simulink model "grid_afe_n"  (R2026a)
settings: Solver=ode23tb  StopTime=simlength  FixedStep=tc  MaxStep=glb_time.tc
values from neighbouring files (symbols this model uses):
  afe_ctrl = ctrl_afe_setup(glb_time.ts_afe, grid_emu.omega_grid_nom)    [init_model.m]
  afe_pwm_phase_shift_mod1 = 0    [init_model.m]
  afe_pwm_phase_shift_mod2 = 0    [init_model.m]
  afe_pwm_phase_shift_mod3 = 0    [init_model.m]
  afe_pwm_phase_shift_mod4 = 0    [init_model.m]
  filters = setup_global_filters(glb_time.ts_afe, glb_time.ts_inv, glb_time.ts_dab, glb_time.tc)    [init_model.m]
  frt_data = frt_settings(test_index, test_subindex, asymmetric_error_type,      enable_frt_1, enable_frt_2, start_time_LVRT, deepPOSxi, deepPOSeta, deepNEGxi, deepNEGeta)    [init_model.m]
  glb_time = timing_setup(fpwm_afe, trgo_afe, fpwm_inv, trgo_inv, fpwm_single_phase_inv, trgo_single_phase_inv, fpwm_dab, trgo_dab,      fpwm_psfbc, trgo_psfbc, fpwm_isop_rail, trgo_isop_rail, fpwm_cllc, trgo_cllc, t_measure, tc_factor, tc_decimation, delay_pwm, dead_time_afe,      dead_time_inv, dead_time_single_phase_inv, dead_time_dab, dead_time_psfbc, dead_time_isop_rail, dead_time_cllc)    [init_model.m]
  grid_emu = grid_three_phase_emulator('Dyn11', delta_star, grid_nominal_power, application_voltage, us1, us2, fgrid,                  eq_grid_inductance, eq_grid_resistance, eta, ucc, i1m, p_iron, n1, n2, core_area, core_length, mur,                  up_xi_pu_ref, up_eta_pu_ref, un_xi_pu_ref, un_eta_pu_ref)    [init_model.m]
  i_react_pos_ref_2 = -ixi_ref_mod1*tan(acos(0.95))    [init_model.m]
  i_react_pos_ref_3 = ixi_ref_mod1*tan(acos(0.95))    [init_model.m]
  ixi_ref_mod1 = -0.85    [init_model.m]
  ixi_ref_mod2 = -0.85    [init_model.m]
  ixi_ref_mod3 = -0.85    [init_model.m]
  ixi_ref_mod4 = -0.85    [init_model.m]
  ki_align = 18    [init_model.m]
  kp_align = 0.25    [init_model.m]
  lim_down_align = -0.05    [init_model.m]
  lim_up_align = 0.05    [init_model.m]
  mavarage_filter_frequency_base_order = 2    [init_model.m]
  time_gain_afe_module_1 = 1.0002    [init_model.m]
  time_gain_afe_module_2 = 1.0015    [init_model.m]
  time_gain_afe_module_3 = 0.9988    [init_model.m]
  time_gain_afe_module_4 = 1.0020    (= 1.002)    [init_model.m]
  time_i_react_pos_ref_1 = start_time_LVRT + error_length + 0.335    [init_model.m]
  time_i_react_pos_ref_2 = time_i_react_pos_ref_1 + 0.5    (= 0.5)    [init_model.m]
  u_cm_comp_mod1 = 0    [init_model.m]
  u_cm_comp_mod2 = -1    [init_model.m]
  u_cm_comp_mod3 = -1    [init_model.m]
  u_cm_comp_mod4 = -1    [init_model.m]
undefined symbols (not defined in the file or in its folder): hwdata, magnitude
libraries: fl_lib x113, nesl_utility x75, moving_average_filter x40, moving_average_filter_cc x32, sl_discontinuities x12, linear_double_integrator_observer_ccaller x8, discrete_time_low_pass_filter x4, threephase_inductor_lib x4, dclink_for_two_levels x4, three_phase_pwm_modulator x4, three_phase_inverter_ideal_switch_based_model x4, three_phase_inverter_igbt_advanced_thermal_model x4
(part 15 of 19)

== system grid_afe_n/afe_abc_mod1/AFE_control/afe_control/current_ctrl/inner_current_ctrl/zero_current_ctrl/zero_sequence_current_ctrl ==
  iz : Inport
  1/Ti : Gain  Gain=afe_ctrl.kp_is_z  SaturateOnIntegerOverflow=on  OutDataTypeStr=Inherit: Same as input  ParamDataTypeStr=Inherit: Same as input
  Constant1 : Constant  Value=0
  Gain : Gain
  Saturation : Saturate  UpperLimit=1  LowerLimit=-1
  Sum1 : Sum  Inputs=+++  SaturateOnIntegerOverflow=on
  Sum2 : Sum  Inputs=-+  SaturateOnIntegerOverflow=on
  Sum3 : Sum  Inputs=-+  SaturateOnIntegerOverflow=on
  Unit Delay4 : UnitDelay  SampleTime=-1
  iz_tracking : Scope  NumInputPorts=3
      settings: ActiveDisplayYMinimum=-1  ActiveDisplayYMaximum=1  DataLoggingVariableName=ScopeData8
  kp : Gain  Gain=afe_ctrl.ki_is_z*glb_time.ts_afe  SaturateOnIntegerOverflow=on  OutDataTypeStr=Inherit: Same as input  ParamDataTypeStr=Inherit: Same as input
  ugamma_afe : Outport
  tag scope: iz_ctrl_out=scoped, iz_pu=scoped, iz_pu_ref=scoped
  wires:
  1/Ti/1 -> Sum1/1, Sum3/1
  kp/1 -> Sum1/2
  Sum3/1 -> Unit Delay4/1
  Unit Delay4/1 -> Sum1/3
  Constant1/1 -> [iz_pu_ref], iz_tracking/1, Sum2/2  "iz_pu_ref"
  iz/1 -> [iz_pu], iz_tracking/2, Sum2/1  "iz_pu"
  Sum2/1 -> kp/1, 1/Ti/1
  Sum1/1 -> Saturation/1
  Saturation/1 -> Gain/1, [iz_ctrl_out], iz_tracking/3, Sum3/2  "iz_ctrl_out"
  Gain/1 -> ugamma_afe/1

== system grid_afe_n/afe_abc_mod1/AFE_control/afe_control/grid_voltage_phase_lock_loops/FHT-PLL/pll_stageA/filter_and_transformation ==
  ug_a : Inport
  ug_b : Inport  Port=2
  ug_c : Inport  Port=3
  Bus Creator : BusCreator  Inputs=2
  Bus Creator1 : BusCreator  Inputs=3
  Bus Creator2 : BusCreator  Inputs=2
  Bus Creator3 : BusCreator  Inputs=3
  Bus Creator4 : BusCreator  Inputs=3
  FHTalpha : Subsystem
  FHTbeta : Subsystem
  FHTdqPLL : Scope  NumInputPorts=2
      settings: ActiveDisplayYMinimum=-1.5258214459194912  ActiveDisplayYMaximum=1.5258228058860459  DataLoggingVariableName=ScopeData12
  Gain : Gain  Gain=-1/2
  Gain1 : Gain  Gain=-1/2
  Sum : Sum  Inputs=|++
  Sum1 : Sum  Inputs=-+|
  To Workspace1 : ToWorkspace  VariableName=ugd_alpha_sim  SampleTime=-1
      settings: MaxDataPoints=glb_time.Ns_afe
  To Workspace2 : ToWorkspace  VariableName=ugd_beta_sim  SampleTime=-1
      settings: MaxDataPoints=glb_time.Ns_afe
  To Workspace3 : ToWorkspace  VariableName=u_fht_alpha_sim  SampleTime=-1
      settings: MaxDataPoints=glb_time.Ns_afe
  To Workspace4 : ToWorkspace  VariableName=v_fht_alpha_sim  SampleTime=-1
      settings: MaxDataPoints=glb_time.Ns_afe
  To Workspace5 : ToWorkspace  VariableName=u_fhtsr_alpha_sim  SampleTime=-1
      settings: MaxDataPoints=glb_time.Ns_afe
  To Workspace6 : ToWorkspace  VariableName=u_fhtsr_beta_sim  SampleTime=-1
      settings: MaxDataPoints=glb_time.Ns_afe
  To Workspace7 : ToWorkspace  VariableName=u_fht_beta_sim  SampleTime=-1
      settings: MaxDataPoints=glb_time.Ns_afe
  To Workspace8 : ToWorkspace  VariableName=v_fht_beta_sim  SampleTime=-1
      settings: MaxDataPoints=glb_time.Ns_afe
  To Workspace9 : ToWorkspace  VariableName=ugd_abc_grid_sim  SampleTime=-1
      settings: MaxDataPoints=glb_time.Ns_afe
  abc2alphabeta : MATLAB Function  TreatAsAtomicUnit=on
  grid_voltages : Scope  NumInputPorts=3
      settings: ActiveDisplayYMinimum=-1.3618303835391998  ActiveDisplayYMaximum=1.3331545889377594  DataLoggingVariableName=ScopeData13
  ug_alpha : Outport  VectorParamsAs1DForOutWhenUnconnected=off
  ug_beta : Outport  Port=2  VectorParamsAs1DForOutWhenUnconnected=off
  wires:
  ug_b/1 -> Bus Creator3/2, grid_voltages/2, abc2alphabeta/2(b)  "ugd_b"
  ug_c/1 -> Bus Creator3/3, grid_voltages/3, abc2alphabeta/3(c)  "ugd_c"
  ug_a/1 -> Bus Creator3/1, grid_voltages/1, abc2alphabeta/1(a)  "ugd_a"
  abc2alphabeta/1(alpha) -> To Workspace1/1, FHTalpha/1(u), Bus Creator4/1  "u_grid_alpha"
  abc2alphabeta/2(beta) -> FHTbeta/1(u), To Workspace2/1, Bus Creator1/1  "u_grid_beta"
  FHTalpha/1(ud_hat) -> To Workspace3/1, Bus Creator/1, Sum/1  "u_fht_alpha"
  Sum/1 -> Gain/1
  FHTbeta/1(ud_hat) -> Sum1/2, To Workspace7/1, Bus Creator2/1  "u_fht_beta"
  Sum1/1 -> Gain1/1
  Gain1/1 -> Bus Creator1/3, To Workspace6/1, ug_beta/1  "u_fhtsr_beta"
  Gain/1 -> Bus Creator4/3, To Workspace5/1, ug_alpha/1  "u_fhtsr_alpha"
  FHTbeta/2(uq_hat) -> Sum/2, To Workspace8/1, Bus Creator2/2  "v_fht_beta"
  FHTalpha/2(uq_hat) -> Sum1/1, To Workspace4/1, Bus Creator/2  "v_fht_alpha"
  Bus Creator1/1 -> FHTdqPLL/2
  Bus Creator4/1 -> FHTdqPLL/1
  Bus Creator/1 -> Bus Creator4/2  "FHTalpha"
  Bus Creator2/1 -> Bus Creator1/2  "FHTbeta"
  Bus Creator3/1 -> To Workspace9/1

== system grid_afe_n/afe_abc_mod1/AFE_control/afe_control/grid_voltage_phase_lock_loops/FHT-PLL/pll_stageA/sequences ==
  u_grid_alpha : Inport
  u_grid_beta : Inport  Port=2
  phase_angle : Inport  Port=3
  alphabeta2xieta : MATLAB Function  TreatAsAtomicUnit=on
  u_grid_xi : Outport
  u_grid_eta : Outport  Port=2
  wires:
  alphabeta2xieta/1(xi) -> u_grid_xi/1  "u_grid_xi"
  alphabeta2xieta/2(eta) -> u_grid_eta/1  "u_grid_eta"
  u_grid_alpha/1 -> alphabeta2xieta/1(alpha)  "u_grid_alpha"
  u_grid_beta/1 -> alphabeta2xieta/2(beta)  "u_grid_beta"
  phase_angle/1 -> alphabeta2xieta/3(gamma)  "phase_angle"

== system grid_afe_n/afe_abc_mod1/AFE_control/afe_control/grid_voltage_phase_lock_loops/FHT-PLL/pll_stageB/double_integrator_observer ==
  theta : Inport
  Gain : Gain  Gain=afe_ctrl.di_obs.Ldso  Multiplication=Matrix(K*u)
  Gain1 : Gain  Gain=afe_ctrl.di_obs.Adso  Multiplication=Matrix(K*u)
  Gain2 : Gain  Gain=afe_ctrl.di_obs.Cso  Multiplication=Matrix(K*u)
  Selector : Selector  InputPortWidth=2  IndexOptions=Index vector (dialog)  Indices=2  OutputSizes=1
  Sum : Sum  Inputs=-+|
  Sum1 : Sum  Inputs=|++
  Unit Delay : UnitDelay  SampleTime=-1
  bounder1 : MATLAB Function  TreatAsAtomicUnit=on
  bounder2 : MATLAB Function  TreatAsAtomicUnit=on
  omega_hat : Outport
  wires:
  Gain/1 -> Sum1/1
  Selector/1 -> omega_hat/1
  Gain2/1 -> bounder2/1(u)  "theta_hat"
  Gain1/1 -> Sum1/2
  Sum1/1 -> Unit Delay/1
  Sum/1 -> bounder1/1(u)  "e"
  Unit Delay/1 -> Gain1/1, Selector/1, Gain2/1
  theta/1 -> Sum/2  "theta"
  bounder1/1(y) -> Gain/1
  bounder2/1(y) -> Sum/1  "theta_hat_bounded"

== system grid_afe_n/afe_abc_mod1/AFE_control/afe_control/grid_voltage_phase_lock_loops/FHT-PLL_simulink/pll_stageA/filter_and_transformation ==
  ug_a : Inport
  ug_b : Inport  Port=2
  ug_c : Inport  Port=3
  Bus Creator : BusCreator  Inputs=2
  Bus Creator1 : BusCreator  Inputs=3
  Bus Creator2 : BusCreator  Inputs=2
  Bus Creator4 : BusCreator  Inputs=3
  FHTalpha : Subsystem
  FHTbeta : Subsystem
  FHTdqPLL : Scope  NumInputPorts=2
      settings: ActiveDisplayYMinimum=-1.5258214459194912  ActiveDisplayYMaximum=1.5258228058860459  DataLoggingVariableName=ScopeData12
  Gain : Gain  Gain=-1/2
  Gain1 : Gain  Gain=-1/2
  Sum : Sum  Inputs=|++
  Sum1 : Sum  Inputs=-+|
  abc2alphabeta : MATLAB Function  TreatAsAtomicUnit=on
  grid_voltages : Scope  NumInputPorts=3
      settings: ActiveDisplayYMinimum=-1.3618303835391998  ActiveDisplayYMaximum=1.3331545889377594  DataLoggingVariableName=ScopeData13
  ug_alpha : Outport  VectorParamsAs1DForOutWhenUnconnected=off
  ug_beta : Outport  Port=2  VectorParamsAs1DForOutWhenUnconnected=off
  wires:
  Bus Creator2/1 -> Bus Creator1/2  "FHTbeta"
  Bus Creator/1 -> Bus Creator4/2  "FHTalpha"
  Bus Creator4/1 -> FHTdqPLL/1
  Bus Creator1/1 -> FHTdqPLL/2
  FHTalpha/2(ubeta) -> Bus Creator/2, Sum1/1  "v_fht_alpha"
  FHTbeta/2(ubeta) -> Bus Creator2/2, Sum/2  "v_fht_beta"
  Gain/1 -> ug_alpha/1, Bus Creator4/3  "u_fhtsr_alpha"
  Gain1/1 -> ug_beta/1, Bus Creator1/3  "u_fhtsr_beta"
  Sum1/1 -> Gain1/1
  FHTbeta/1(ualpha) -> Bus Creator2/1, Sum1/2  "u_fht_beta"
  Sum/1 -> Gain/1
  FHTalpha/1(ualpha) -> Sum/1, Bus Creator/1  "u_fht_alpha"
  abc2alphabeta/2(beta) -> FHTbeta/1(u), Bus Creator1/1  "u_grid_beta"
  abc2alphabeta/1(alpha) -> FHTalpha/1(u), Bus Creator4/1  "u_grid_alpha"
  ug_a/1 -> abc2alphabeta/1(a), grid_voltages/1  "ugd_a"
  ug_c/1 -> abc2alphabeta/3(c), grid_voltages/3  "ugd_c"
  ug_b/1 -> abc2alphabeta/2(b), grid_voltages/2  "ugd_b"

== system grid_afe_n/afe_abc_mod1/AFE_control/afe_control/grid_voltage_phase_lock_loops/FHT-PLL_simulink/pll_stageA/sequences ==
  u_grid_alpha : Inport
  u_grid_beta : Inport  Port=2
  phase_angle : Inport  Port=3
  alphabeta2xieta : MATLAB Function  TreatAsAtomicUnit=on
  u_grid_xi : Outport
  u_grid_eta : Outport  Port=2
  wires:
  phase_angle/1 -> alphabeta2xieta/3(gamma)  "phase_angle"
  u_grid_beta/1 -> alphabeta2xieta/2(beta)  "u_grid_beta"
  u_grid_alpha/1 -> alphabeta2xieta/1(alpha)  "u_grid_alpha"
  alphabeta2xieta/2(eta) -> u_grid_eta/1  "u_grid_eta"
  alphabeta2xieta/1(xi) -> u_grid_xi/1  "u_grid_xi"

== system grid_afe_n/afe_abc_mod1/AFE_control/afe_control/grid_voltage_phase_lock_loops/FHT-PLL_simulink/pll_stageB/double_integrator_observer ==
  theta : Inport
  Gain : Gain  Gain=afe_ctrl.di_obs.Ldso  Multiplication=Matrix(K*u)
  Gain1 : Gain  Gain=afe_ctrl.di_obs.Adso  Multiplication=Matrix(K*u)
  Gain2 : Gain  Gain=afe_ctrl.di_obs.Cso  Multiplication=Matrix(K*u)
  Selector : Selector  InputPortWidth=2  IndexOptions=Index vector (dialog)  Indices=2  OutputSizes=1
  Sum : Sum  Inputs=-+|
  Sum1 : Sum  Inputs=|++
  Unit Delay : UnitDelay  SampleTime=-1
  bounder1 : MATLAB Function  TreatAsAtomicUnit=on
  bounder2 : MATLAB Function  TreatAsAtomicUnit=on
  omega_hat : Outport
  wires:
  bounder2/1(y) -> Sum/1  "theta_hat_bounded"
  bounder1/1(y) -> Gain/1
  theta/1 -> Sum/2  "theta"
  Unit Delay/1 -> Gain2/1, Selector/1, Gain1/1
  Sum/1 -> bounder1/1(u)  "e"
  Sum1/1 -> Unit Delay/1
  Gain1/1 -> Sum1/2
  Gain2/1 -> bounder2/1(u)  "theta_hat"
  Selector/1 -> omega_hat/1
  Gain/1 -> Sum1/1

== system grid_afe_n/afe_abc_mod1/AFE_control/afe_control/grid_voltage_phase_lock_loops/dq_pll/pll_stageA/mormalization_and_transformation ==
  ug_a : Inport
  ug_b : Inport  Port=2
  ug_c : Inport  Port=3
  abc2alphabeta : MATLAB Function  TreatAsAtomicUnit=on
  ug_alpha : Outport  VectorParamsAs1DForOutWhenUnconnected=off
  ug_beta : Outport  Port=2  VectorParamsAs1DForOutWhenUnconnected=off
  wires:
  abc2alphabeta/2(beta) -> ug_beta/1  "u_grid_beta"
  abc2alphabeta/1(alpha) -> ug_alpha/1  "u_grid_alpha"
  ug_a/1 -> abc2alphabeta/1(a)
  ug_b/1 -> abc2alphabeta/2(b)
  ug_c/1 -> abc2alphabeta/3(c)

== system grid_afe_n/afe_abc_mod1/AFE_control/afe_control/grid_voltage_phase_lock_loops/dq_pll/pll_stageA/sequences ==
  u_grid_alpha : Inport
  u_grid_beta : Inport  Port=2
  gamma_grid : Inport  Port=3
  Terminator : Terminator
  Terminator1 : Terminator
  alphabeta2xieta : Subsystem
  u_grid_pos_xi : Outport
  u_grid_pos_eta : Outport  Port=2
  wires:
  alphabeta2xieta/1(xi) -> u_grid_pos_xi/1  "u_grid_pos_xi"
  alphabeta2xieta/2(eta) -> u_grid_pos_eta/1  "u_grid_pos_eta"
  u_grid_alpha/1 -> alphabeta2xieta/1(alpha)  "u_grid_alpha"
  u_grid_beta/1 -> alphabeta2xieta/2(beta)  "u_grid_beta"
  gamma_grid/1 -> alphabeta2xieta/3(gamma)  "phase_grid"
  alphabeta2xieta/3(Out3) -> Terminator/1  "neg_xi"
  alphabeta2xieta/4(Out4) -> Terminator1/1  "neg_eta"

== system grid_afe_n/afe_abc_mod1/AFE_control/afe_control/grid_voltage_phase_lock_loops/dq_pll/pll_stageB/double_integrator_observer ==
  phase : Inport
  Gain : Gain  Gain=afe_ctrl.di_obs.Ldso  Multiplication=Matrix(K*u)
  Gain1 : Gain  Gain=afe_ctrl.di_obs.Adso  Multiplication=Matrix(K*u)
  Gain2 : Gain  Gain=afe_ctrl.di_obs.Cso  Multiplication=Matrix(K*u)
  Selector : Selector  InputPortWidth=2  IndexOptions=Index vector (dialog)  Indices=2  OutputSizes=1
  Sum : Sum  Inputs=-+|
  Sum1 : Sum  Inputs=|++
  Unit Delay : UnitDelay  SampleTime=-1
  bounder1 : MATLAB Function  TreatAsAtomicUnit=on
  bounder2 : MATLAB Function  TreatAsAtomicUnit=on
  omega_hat : Outport
  wires:
  Gain/1 -> Sum1/1
  Selector/1 -> omega_hat/1
  Gain2/1 -> bounder2/1(u)  "theta_hat"
  Gain1/1 -> Sum1/2
  Sum1/1 -> Unit Delay/1
  Sum/1 -> bounder1/1(u)  "e"
  Unit Delay/1 -> Gain1/1, Selector/1, Gain2/1
  phase/1 -> Sum/2  "phase"
  bounder1/1(y) -> Gain/1  "e_bounded"
  bounder2/1(y) -> Sum/1  "theta_hat_bounded"

== system grid_afe_n/afe_abc_mod1/AFE_control/afe_control/grid_voltage_phase_lock_loops/dq_pll/pll_stageB/scheduled-p-gain ==
  In1 : Inport
  Switch : Switch  Criteria=u2 > Threshold  Threshold=0.5  SaturateOnIntegerOverflow=off  InputSameDT=off
  kp1 : Gain  Gain=afe_ctrl.pll_p  SaturateOnIntegerOverflow=on  OutDataTypeStr=Inherit: Same as input  ParamDataTypeStr=Inherit: Same as input
  kp3 : Gain  Gain=afe_ctrl.pll_p_frt  SaturateOnIntegerOverflow=on  OutDataTypeStr=Inherit: Same as input  ParamDataTypeStr=Inherit: Same as input
  Out2 : Outport
  wires:
  kp3/1 -> Switch/1
  kp1/1 -> Switch/3
  [frt_active] -> Switch/2
  In1/1 -> kp1/1, kp3/1
  Switch/1 -> Out2/1

== system grid_afe_n/afe_abc_mod2/AFE_control/afe_control/current_ctrl/inner_current_ctrl/zero_current_ctrl/antiwind_up ==
  d_abc : Inport
  Add : Sum
  Bus Creator : BusCreator  Inputs=3
  Constant : Constant  Value=0
  Demux1 : Demux  Outputs=3
  MATLAB Function1 : MATLAB Function  TreatAsAtomicUnit=on
  MATLAB Function2 : MATLAB Function  TreatAsAtomicUnit=on
  Terminator : Terminator
  Unit Delay1 : UnitDelay  SampleTime=-1
  Unit Delay4 : UnitDelay  SampleTime=-1
  Unit Delay5 : UnitDelay  SampleTime=-1
  afe_ictrl_out/afe_ictrl_ff : Scope  NumInputPorts=3
      settings: ActiveDisplayYMinimum=-1.3378870671178225  ActiveDisplayYMaximum=1.3487234823223584  DataLoggingVariableName=ScopeData4
  anti_wind_up : Subsystem
  ualpha_afe : Outport
  ubeta_afe : Outport  Port=2
  wires:
  Constant/1 -> Add/2
  MATLAB Function2/3(gamma) -> Terminator/1  "u_gamma"
  Unit Delay5/1 -> ubeta_afe/1, anti_wind_up/2(beta)  "ubeta_afe"
  MATLAB Function2/2(beta) -> Unit Delay5/1  "u_beta"
  Unit Delay4/1 -> ualpha_afe/1, anti_wind_up/1(alpha)  "ualpha_afe"
  MATLAB Function2/1(alpha) -> Unit Delay4/1  "u_alpha"
  MATLAB Function1/2(dbs) -> Bus Creator/2, MATLAB Function2/2(b)  "dbs"
  Add/1 -> Demux1/1  "d_abc_sum"
  Demux1/1 -> MATLAB Function1/1(da)  "da"
  anti_wind_up/1(scaling) -> MATLAB Function1/4(scaling)
  Unit Delay1/1 -> afe_ictrl_out/afe_ictrl_ff/3  "u_grid_ff_abc_mod1"
  Bus Creator/1 -> afe_ictrl_out/afe_ictrl_ff/1  "ds_abc"
  Demux1/3 -> MATLAB Function1/3(dc)  "dc"
  Demux1/2 -> MATLAB Function1/2(db)  "db"
  [v_grid_ff_abc] -> Unit Delay1/1
  MATLAB Function1/3(dcs) -> Bus Creator/3, MATLAB Function2/3(c)  "dcs"
  d_abc/1 -> afe_ictrl_out/afe_ictrl_ff/2, Add/1
  MATLAB Function1/1(das) -> Bus Creator/1, MATLAB Function2/1(a)  "das"

== system grid_afe_n/afe_abc_mod2/AFE_control/afe_control/current_ctrl/inner_current_ctrl/zero_current_ctrl/iz ==
  Demux : Demux  Outputs=3
  Gain : Gain  Gain=1/3
  Sum : Sum  Inputs=+++
  iz : Outport
  wires:
  Gain/1 -> iz/1
  Demux/2 -> Sum/2  "is_b"
  Demux/3 -> Sum/3  "is_c"
  [isd_abc_pu] -> Demux/1
  Demux/1 -> Sum/1  "is_a"
  Sum/1 -> Gain/1

== system grid_afe_n/afe_abc_mod2/AFE_control/afe_control/current_ctrl/inner_current_ctrl/zero_current_ctrl/zero_sequence_current_ctrl ==
  iz : Inport
  1/Ti : Gain  Gain=afe_ctrl.kp_is_z  SaturateOnIntegerOverflow=on  OutDataTypeStr=Inherit: Same as input  ParamDataTypeStr=Inherit: Same as input
  Constant1 : Constant  Value=0
  Gain : Gain
  Saturation : Saturate  UpperLimit=1  LowerLimit=-1
  Sum1 : Sum  Inputs=+++  SaturateOnIntegerOverflow=on
  Sum2 : Sum  Inputs=-+  SaturateOnIntegerOverflow=on
  Sum3 : Sum  Inputs=-+  SaturateOnIntegerOverflow=on
  Unit Delay4 : UnitDelay  SampleTime=-1
  iz_tracking : Scope  NumInputPorts=3
      settings: ActiveDisplayYMinimum=-1  ActiveDisplayYMaximum=1  DataLoggingVariableName=ScopeData8
  kp : Gain  Gain=afe_ctrl.ki_is_z*glb_time.ts_afe  SaturateOnIntegerOverflow=on  OutDataTypeStr=Inherit: Same as input  ParamDataTypeStr=Inherit: Same as input
  ugamma_afe : Outport
  tag scope: iz_ctrl_out=scoped, iz_pu=scoped, iz_pu_ref=scoped
  wires:
  Gain/1 -> ugamma_afe/1
  Saturation/1 -> Sum3/2, iz_tracking/3, [iz_ctrl_out], Gain/1  "iz_ctrl_out"
  Sum1/1 -> Saturation/1
  Sum2/1 -> 1/Ti/1, kp/1
  iz/1 -> Sum2/1, iz_tracking/2, [iz_pu]  "iz_pu"
  Constant1/1 -> Sum2/2, iz_tracking/1, [iz_pu_ref]  "iz_pu_ref"
  Unit Delay4/1 -> Sum1/3
  Sum3/1 -> Unit Delay4/1
  kp/1 -> Sum1/2
  1/Ti/1 -> Sum3/1, Sum1/1

== system grid_afe_n/afe_abc_mod2/AFE_control/afe_control/grid_voltage_phase_lock_loops/FHT-PLL/pll_stageA/filter_and_transformation ==
  ug_a : Inport
  ug_b : Inport  Port=2
  ug_c : Inport  Port=3
  Bus Creator : BusCreator  Inputs=2
  Bus Creator1 : BusCreator  Inputs=3
  Bus Creator2 : BusCreator  Inputs=2
  Bus Creator3 : BusCreator  Inputs=3
  Bus Creator4 : BusCreator  Inputs=3
  FHTalpha : Subsystem
  FHTbeta : Subsystem
  FHTdqPLL : Scope  NumInputPorts=2
      settings: ActiveDisplayYMinimum=-1.5258214459194912  ActiveDisplayYMaximum=1.5258228058860459  DataLoggingVariableName=ScopeData12
  Gain : Gain  Gain=-1/2
  Gain1 : Gain  Gain=-1/2
  Sum : Sum  Inputs=|++
  Sum1 : Sum  Inputs=-+|
  To Workspace1 : ToWorkspace  VariableName=ugd_alpha_sim  SampleTime=-1
      settings: MaxDataPoints=glb_time.Ns_afe
  To Workspace2 : ToWorkspace  VariableName=ugd_beta_sim  SampleTime=-1
      settings: MaxDataPoints=glb_time.Ns_afe
  To Workspace3 : ToWorkspace  VariableName=u_fht_alpha_sim  SampleTime=-1
      settings: MaxDataPoints=glb_time.Ns_afe
  To Workspace4 : ToWorkspace  VariableName=v_fht_alpha_sim  SampleTime=-1
      settings: MaxDataPoints=glb_time.Ns_afe
  To Workspace5 : ToWorkspace  VariableName=u_fhtsr_alpha_sim  SampleTime=-1
      settings: MaxDataPoints=glb_time.Ns_afe
  To Workspace6 : ToWorkspace  VariableName=u_fhtsr_beta_sim  SampleTime=-1
      settings: MaxDataPoints=glb_time.Ns_afe
  To Workspace7 : ToWorkspace  VariableName=u_fht_beta_sim  SampleTime=-1
      settings: MaxDataPoints=glb_time.Ns_afe
  To Workspace8 : ToWorkspace  VariableName=v_fht_beta_sim  SampleTime=-1
      settings: MaxDataPoints=glb_time.Ns_afe
  To Workspace9 : ToWorkspace  VariableName=ugd_abc_grid_sim  SampleTime=-1
      settings: MaxDataPoints=glb_time.Ns_afe
  abc2alphabeta : MATLAB Function  TreatAsAtomicUnit=on
  grid_voltages : Scope  NumInputPorts=3
      settings: ActiveDisplayYMinimum=-1.3618303835391998  ActiveDisplayYMaximum=1.3331545889377594  DataLoggingVariableName=ScopeData13
  ug_alpha : Outport  VectorParamsAs1DForOutWhenUnconnected=off
  ug_beta : Outport  Port=2  VectorParamsAs1DForOutWhenUnconnected=off
  wires:
  Bus Creator3/1 -> To Workspace9/1
  Bus Creator2/1 -> Bus Creator1/2  "FHTbeta"
  Bus Creator/1 -> Bus Creator4/2  "FHTalpha"
  Bus Creator4/1 -> FHTdqPLL/1
  Bus Creator1/1 -> FHTdqPLL/2
  FHTalpha/2(uq_hat) -> Bus Creator/2, To Workspace4/1, Sum1/1  "v_fht_alpha"
  FHTbeta/2(uq_hat) -> Bus Creator2/2, To Workspace8/1, Sum/2  "v_fht_beta"
  Gain/1 -> ug_alpha/1, To Workspace5/1, Bus Creator4/3  "u_fhtsr_alpha"
  Gain1/1 -> ug_beta/1, To Workspace6/1, Bus Creator1/3  "u_fhtsr_beta"
  Sum1/1 -> Gain1/1
  FHTbeta/1(ud_hat) -> Bus Creator2/1, To Workspace7/1, Sum1/2  "u_fht_beta"
  Sum/1 -> Gain/1
  FHTalpha/1(ud_hat) -> Sum/1, Bus Creator/1, To Workspace3/1  "u_fht_alpha"
  abc2alphabeta/2(beta) -> Bus Creator1/1, To Workspace2/1, FHTbeta/1(u)  "u_grid_beta"
  abc2alphabeta/1(alpha) -> Bus Creator4/1, FHTalpha/1(u), To Workspace1/1  "u_grid_alpha"
  ug_a/1 -> abc2alphabeta/1(a), grid_voltages/1, Bus Creator3/1  "ugd_a"
  ug_c/1 -> abc2alphabeta/3(c), grid_voltages/3, Bus Creator3/3  "ugd_c"
  ug_b/1 -> abc2alphabeta/2(b), grid_voltages/2, Bus Creator3/2  "ugd_b"

== system grid_afe_n/afe_abc_mod2/AFE_control/afe_control/grid_voltage_phase_lock_loops/FHT-PLL/pll_stageA/sequences ==
  u_grid_alpha : Inport
  u_grid_beta : Inport  Port=2
  phase_angle : Inport  Port=3
  alphabeta2xieta : MATLAB Function  TreatAsAtomicUnit=on
  u_grid_xi : Outport
  u_grid_eta : Outport  Port=2
  wires:
  phase_angle/1 -> alphabeta2xieta/3(gamma)  "phase_angle"
  u_grid_beta/1 -> alphabeta2xieta/2(beta)  "u_grid_beta"
  u_grid_alpha/1 -> alphabeta2xieta/1(alpha)  "u_grid_alpha"
  alphabeta2xieta/2(eta) -> u_grid_eta/1  "u_grid_eta"
  alphabeta2xieta/1(xi) -> u_grid_xi/1  "u_grid_xi"

== system grid_afe_n/afe_abc_mod2/AFE_control/afe_control/grid_voltage_phase_lock_loops/FHT-PLL/pll_stageB/double_integrator_observer ==
  theta : Inport
  Gain : Gain  Gain=afe_ctrl.di_obs.Ldso  Multiplication=Matrix(K*u)
  Gain1 : Gain  Gain=afe_ctrl.di_obs.Adso  Multiplication=Matrix(K*u)
  Gain2 : Gain  Gain=afe_ctrl.di_obs.Cso  Multiplication=Matrix(K*u)
  Selector : Selector  InputPortWidth=2  IndexOptions=Index vector (dialog)  Indices=2  OutputSizes=1
  Sum : Sum  Inputs=-+|
  Sum1 : Sum  Inputs=|++
  Unit Delay : UnitDelay  SampleTime=-1
  bounder1 : MATLAB Function  TreatAsAtomicUnit=on
  bounder2 : MATLAB Function  TreatAsAtomicUnit=on
  omega_hat : Outport
  wires:
  bounder2/1(y) -> Sum/1  "theta_hat_bounded"
  bounder1/1(y) -> Gain/1
  theta/1 -> Sum/2  "theta"
  Unit Delay/1 -> Gain2/1, Selector/1, Gain1/1
  Sum/1 -> bounder1/1(u)  "e"
  Sum1/1 -> Unit Delay/1
  Gain1/1 -> Sum1/2
  Gain2/1 -> bounder2/1(u)  "theta_hat"
  Selector/1 -> omega_hat/1
  Gain/1 -> Sum1/1

== system grid_afe_n/afe_abc_mod2/AFE_control/afe_control/grid_voltage_phase_lock_loops/FHT-PLL_simulink/pll_stageA/filter_and_transformation ==
  ug_a : Inport
  ug_b : Inport  Port=2
  ug_c : Inport  Port=3
  Bus Creator : BusCreator  Inputs=2
  Bus Creator1 : BusCreator  Inputs=3
  Bus Creator2 : BusCreator  Inputs=2
  Bus Creator4 : BusCreator  Inputs=3
  FHTalpha : Subsystem
  FHTbeta : Subsystem
  FHTdqPLL : Scope  NumInputPorts=2
      settings: ActiveDisplayYMinimum=-1.4370650300424566  ActiveDisplayYMaximum=1.3792236516012133  DataLoggingVariableName=ScopeData12
  Gain : Gain  Gain=-1/2
  Gain1 : Gain  Gain=-1/2
  Sum : Sum  Inputs=|++
  Sum1 : Sum  Inputs=-+|
  abc2alphabeta : MATLAB Function  TreatAsAtomicUnit=on
  grid_voltages : Scope  NumInputPorts=3
      settings: ActiveDisplayYMinimum=-1.3620119839906693  ActiveDisplayYMaximum=1.3591613322496414  DataLoggingVariableName=ScopeData13
  ug_alpha : Outport  VectorParamsAs1DForOutWhenUnconnected=off
  ug_beta : Outport  Port=2  VectorParamsAs1DForOutWhenUnconnected=off
  wires:
  Bus Creator2/1 -> Bus Creator1/2  "FHTbeta"
  Bus Creator/1 -> Bus Creator4/2  "FHTalpha"
  Bus Creator4/1 -> FHTdqPLL/1
  Bus Creator1/1 -> FHTdqPLL/2
  FHTalpha/2(ubeta) -> Bus Creator/2, Sum1/1  "v_fht_alpha"
  FHTbeta/2(ubeta) -> Bus Creator2/2, Sum/2  "v_fht_beta"
  Gain/1 -> ug_alpha/1, Bus Creator4/3  "u_fhtsr_alpha"
  Gain1/1 -> ug_beta/1, Bus Creator1/3  "u_fhtsr_beta"
  Sum1/1 -> Gain1/1
  FHTbeta/1(ualpha) -> Bus Creator2/1, Sum1/2  "u_fht_beta"
  Sum/1 -> Gain/1
  FHTalpha/1(ualpha) -> Sum/1, Bus Creator/1  "u_fht_alpha"
  abc2alphabeta/2(beta) -> FHTbeta/1(u), Bus Creator1/1  "u_grid_beta"
  abc2alphabeta/1(alpha) -> FHTalpha/1(u), Bus Creator4/1  "u_grid_alpha"
  ug_a/1 -> abc2alphabeta/1(a), grid_voltages/1  "ugd_a"
  ug_c/1 -> abc2alphabeta/3(c), grid_voltages/3  "ugd_c"
  ug_b/1 -> abc2alphabeta/2(b), grid_voltages/2  "ugd_b"

== system grid_afe_n/afe_abc_mod2/AFE_control/afe_control/grid_voltage_phase_lock_loops/FHT-PLL_simulink/pll_stageA/sequences ==
  u_grid_alpha : Inport
  u_grid_beta : Inport  Port=2
  phase_angle : Inport  Port=3
  alphabeta2xieta : MATLAB Function  TreatAsAtomicUnit=on
  u_grid_xi : Outport
  u_grid_eta : Outport  Port=2
  wires:
  phase_angle/1 -> alphabeta2xieta/3(gamma)  "phase_angle"
  u_grid_beta/1 -> alphabeta2xieta/2(beta)  "u_grid_beta"
  u_grid_alpha/1 -> alphabeta2xieta/1(alpha)  "u_grid_alpha"
  alphabeta2xieta/2(eta) -> u_grid_eta/1  "u_grid_eta"
  alphabeta2xieta/1(xi) -> u_grid_xi/1  "u_grid_xi"

== system grid_afe_n/afe_abc_mod2/AFE_control/afe_control/grid_voltage_phase_lock_loops/FHT-PLL_simulink/pll_stageB/double_integrator_observer ==
  theta : Inport
  Gain : Gain  Gain=afe_ctrl.di_obs.Ldso  Multiplication=Matrix(K*u)
  Gain1 : Gain  Gain=afe_ctrl.di_obs.Adso  Multiplication=Matrix(K*u)
  Gain2 : Gain  Gain=afe_ctrl.di_obs.Cso  Multiplication=Matrix(K*u)
  Selector : Selector  InputPortWidth=2  IndexOptions=Index vector (dialog)  Indices=2  OutputSizes=1
  Sum : Sum  Inputs=-+|
  Sum1 : Sum  Inputs=|++
  Unit Delay : UnitDelay  SampleTime=-1
  bounder1 : MATLAB Function  TreatAsAtomicUnit=on
  bounder2 : MATLAB Function  TreatAsAtomicUnit=on
  omega_hat : Outport
  wires:
  bounder2/1(y) -> Sum/1  "theta_hat_bounded"
  bounder1/1(y) -> Gain/1
  theta/1 -> Sum/2  "theta"
  Unit Delay/1 -> Gain2/1, Selector/1, Gain1/1
  Sum/1 -> bounder1/1(u)  "e"
  Sum1/1 -> Unit Delay/1
  Gain1/1 -> Sum1/2
  Gain2/1 -> bounder2/1(u)  "theta_hat"
  Selector/1 -> omega_hat/1
  Gain/1 -> Sum1/1

== system grid_afe_n/afe_abc_mod2/AFE_control/afe_control/grid_voltage_phase_lock_loops/dq_pll/pll_stageA/mormalization_and_transformation ==
  ug_a : Inport
  ug_b : Inport  Port=2
  ug_c : Inport  Port=3
  abc2alphabeta : MATLAB Function  TreatAsAtomicUnit=on
  ug_alpha : Outport  VectorParamsAs1DForOutWhenUnconnected=off
  ug_beta : Outport  Port=2  VectorParamsAs1DForOutWhenUnconnected=off
  wires:
  ug_c/1 -> abc2alphabeta/3(c)
  ug_b/1 -> abc2alphabeta/2(b)
  ug_a/1 -> abc2alphabeta/1(a)
  abc2alphabeta/1(alpha) -> ug_alpha/1  "u_grid_alpha"
  abc2alphabeta/2(beta) -> ug_beta/1  "u_grid_beta"

== system grid_afe_n/afe_abc_mod2/AFE_control/afe_control/grid_voltage_phase_lock_loops/dq_pll/pll_stageA/sequences ==
  u_grid_alpha : Inport
  u_grid_beta : Inport  Port=2
  gamma_grid : Inport  Port=3
  alphabeta2xieta : Subsystem
  u_grid_pos_xi : Outport
  u_grid_pos_eta : Outport  Port=2
  wires:
  gamma_grid/1 -> alphabeta2xieta/3(gamma)  "phase_grid"
  u_grid_beta/1 -> alphabeta2xieta/2(beta)  "u_grid_beta"
  u_grid_alpha/1 -> alphabeta2xieta/1(alpha)  "u_grid_alpha"
  alphabeta2xieta/2(eta) -> u_grid_pos_eta/1  "u_grid_pos_eta"
  alphabeta2xieta/1(xi) -> u_grid_pos_xi/1  "u_grid_pos_xi"

== system grid_afe_n/afe_abc_mod2/AFE_control/afe_control/grid_voltage_phase_lock_loops/dq_pll/pll_stageB/double_integrator_observer ==
  phase : Inport
  Gain : Gain  Gain=afe_ctrl.di_obs.Ldso  Multiplication=Matrix(K*u)
  Gain1 : Gain  Gain=afe_ctrl.di_obs.Adso  Multiplication=Matrix(K*u)
  Gain2 : Gain  Gain=afe_ctrl.di_obs.Cso  Multiplication=Matrix(K*u)
  Selector : Selector  InputPortWidth=2  IndexOptions=Index vector (dialog)  Indices=2  OutputSizes=1
  Sum : Sum  Inputs=-+|
  Sum1 : Sum  Inputs=|++
  Unit Delay : UnitDelay  SampleTime=-1
  bounder1 : MATLAB Function  TreatAsAtomicUnit=on
  bounder2 : MATLAB Function  TreatAsAtomicUnit=on
  omega_hat : Outport
  wires:
  bounder2/1(y) -> Sum/1  "theta_hat_bounded"
  bounder1/1(y) -> Gain/1  "e_bounded"
  phase/1 -> Sum/2  "phase"
  Unit Delay/1 -> Gain2/1, Selector/1, Gain1/1
  Sum/1 -> bounder1/1(u)  "e"
  Sum1/1 -> Unit Delay/1
  Gain1/1 -> Sum1/2
  Gain2/1 -> bounder2/1(u)  "theta_hat"
  Selector/1 -> omega_hat/1
  Gain/1 -> Sum1/1

== system grid_afe_n/afe_abc_mod2/AFE_control/afe_control/grid_voltage_phase_lock_loops/dq_pll/pll_stageB/scheduled-p-gain ==
  in : Inport
  Switch : Switch  Criteria=u2 > Threshold  Threshold=0.5  SaturateOnIntegerOverflow=off  InputSameDT=off
  kp1 : Gain  Gain=afe_ctrl.pll_p  SaturateOnIntegerOverflow=on  OutDataTypeStr=Inherit: Same as input  ParamDataTypeStr=Inherit: Same as input
  kp3 : Gain  Gain=afe_ctrl.pll_p_frt  SaturateOnIntegerOverflow=on  OutDataTypeStr=Inherit: Same as input  ParamDataTypeStr=Inherit: Same as input
  out : Outport
  wires:
  Switch/1 -> out/1
  in/1 -> kp3/1, kp1/1
  [frt_active] -> Switch/2
  kp1/1 -> Switch/3
  kp3/1 -> Switch/1

== system grid_afe_n/afe_abc_mod3/AFE_control/afe_control/current_ctrl/inner_current_ctrl/zero_current_ctrl/antiwind_up ==
  d_abc : Inport
  Add : Sum
  Bus Creator : BusCreator  Inputs=3
  Constant : Constant  Value=0
  Demux1 : Demux  Outputs=3
  MATLAB Function1 : MATLAB Function  TreatAsAtomicUnit=on
  MATLAB Function2 : MATLAB Function  TreatAsAtomicUnit=on
  Terminator : Terminator
  Unit Delay1 : UnitDelay  SampleTime=-1
  Unit Delay4 : UnitDelay  SampleTime=-1
  Unit Delay5 : UnitDelay  SampleTime=-1
  afe_ictrl_out/afe_ictrl_ff : Scope  NumInputPorts=3
      settings: ActiveDisplayYMinimum=-2.3644997050526393  ActiveDisplayYMaximum=2.3332899605671109  DataLoggingVariableName=ScopeData4
  anti_wind_up : Subsystem
  ualpha_afe : Outport
  ubeta_afe : Outport  Port=2
  wires:
  MATLAB Function1/1(das) -> MATLAB Function2/1(a), Bus Creator/1  "das"
  d_abc/1 -> Add/1, afe_ictrl_out/afe_ictrl_ff/2
  MATLAB Function1/3(dcs) -> MATLAB Function2/3(c), Bus Creator/3  "dcs"
  [v_grid_ff_abc] -> Unit Delay1/1
  Demux1/2 -> MATLAB Function1/2(db)  "db"
  Demux1/3 -> MATLAB Function1/3(dc)  "dc"
  Bus Creator/1 -> afe_ictrl_out/afe_ictrl_ff/1  "ds_abc"
  Unit Delay1/1 -> afe_ictrl_out/afe_ictrl_ff/3  "u_grid_ff_abc_mod1"
  anti_wind_up/1(scaling) -> MATLAB Function1/4(scaling)
  Demux1/1 -> MATLAB Function1/1(da)  "da"
  Add/1 -> Demux1/1  "d_abc_sum"
  MATLAB Function1/2(dbs) -> MATLAB Function2/2(b), Bus Creator/2  "dbs"
  MATLAB Function2/1(alpha) -> Unit Delay4/1  "u_alpha"
  Unit Delay4/1 -> anti_wind_up/1(alpha), ualpha_afe/1  "ualpha_afe"
  MATLAB Function2/2(beta) -> Unit Delay5/1  "u_beta"
  Unit Delay5/1 -> anti_wind_up/2(beta), ubeta_afe/1  "ubeta_afe"
  MATLAB Function2/3(gamma) -> Terminator/1  "u_gamma"
  Constant/1 -> Add/2

== system grid_afe_n/afe_abc_mod3/AFE_control/afe_control/current_ctrl/inner_current_ctrl/zero_current_ctrl/iz ==
  Demux : Demux  Outputs=3
  Gain : Gain  Gain=1/3
  Sum : Sum  Inputs=+++
  iz : Outport
  wires:
  Sum/1 -> Gain/1
  Demux/1 -> Sum/1  "is_a"
  [isd_abc_pu] -> Demux/1
  Demux/3 -> Sum/3  "is_c"
  Demux/2 -> Sum/2  "is_b"
  Gain/1 -> iz/1

== system grid_afe_n/afe_abc_mod3/AFE_control/afe_control/current_ctrl/inner_current_ctrl/zero_current_ctrl/zero_sequence_current_ctrl ==
  iz : Inport
  1/Ti : Gain  Gain=afe_ctrl.kp_is_z  SaturateOnIntegerOverflow=on  OutDataTypeStr=Inherit: Same as input  ParamDataTypeStr=Inherit: Same as input
  Constant1 : Constant  Value=0
  Gain : Gain
  Saturation : Saturate  UpperLimit=1  LowerLimit=-1
  Sum1 : Sum  Inputs=+++  SaturateOnIntegerOverflow=on
  Sum2 : Sum  Inputs=-+  SaturateOnIntegerOverflow=on
  Sum3 : Sum  Inputs=-+  SaturateOnIntegerOverflow=on
  Unit Delay4 : UnitDelay  SampleTime=-1
  iz_tracking : Scope  NumInputPorts=3
      settings: ActiveDisplayYMinimum=-1  ActiveDisplayYMaximum=1  DataLoggingVariableName=ScopeData8
  kp : Gain  Gain=afe_ctrl.ki_is_z*glb_time.ts_afe  SaturateOnIntegerOverflow=on  OutDataTypeStr=Inherit: Same as input  ParamDataTypeStr=Inherit: Same as input
  ugamma_afe : Outport
  tag scope: iz_ctrl_out=scoped, iz_pu=scoped, iz_pu_ref=scoped
  wires:
  1/Ti/1 -> Sum1/1, Sum3/1
  kp/1 -> Sum1/2
  Sum3/1 -> Unit Delay4/1
  Unit Delay4/1 -> Sum1/3
  Constant1/1 -> [iz_pu_ref], iz_tracking/1, Sum2/2  "iz_pu_ref"
  iz/1 -> [iz_pu], iz_tracking/2, Sum2/1  "iz_pu"
  Sum2/1 -> kp/1, 1/Ti/1
  Sum1/1 -> Saturation/1
  Saturation/1 -> Gain/1, [iz_ctrl_out], iz_tracking/3, Sum3/2  "iz_ctrl_out"
  Gain/1 -> ugamma_afe/1

== system grid_afe_n/afe_abc_mod3/AFE_control/afe_control/grid_voltage_phase_lock_loops/FHT-PLL/pll_stageA/filter_and_transformation ==
  ug_a : Inport
  ug_b : Inport  Port=2
  ug_c : Inport  Port=3
  Bus Creator : BusCreator  Inputs=2
  Bus Creator1 : BusCreator  Inputs=3
  Bus Creator2 : BusCreator  Inputs=2
  Bus Creator3 : BusCreator  Inputs=3
  Bus Creator4 : BusCreator  Inputs=3
  FHTalpha : Subsystem
  FHTbeta : Subsystem
  FHTdqPLL : Scope  NumInputPorts=2
      settings: ActiveDisplayYMinimum=-1.5258214459194912  ActiveDisplayYMaximum=1.5258228058860459  DataLoggingVariableName=ScopeData12
  Gain : Gain  Gain=-1/2
  Gain1 : Gain  Gain=-1/2
  Sum : Sum  Inputs=|++
  Sum1 : Sum  Inputs=-+|
  To Workspace1 : ToWorkspace  VariableName=ugd_alpha_sim  SampleTime=-1
      settings: MaxDataPoints=glb_time.Ns_afe
  To Workspace2 : ToWorkspace  VariableName=ugd_beta_sim  SampleTime=-1
      settings: MaxDataPoints=glb_time.Ns_afe
  To Workspace3 : ToWorkspace  VariableName=u_fht_alpha_sim  SampleTime=-1
      settings: MaxDataPoints=glb_time.Ns_afe
  To Workspace4 : ToWorkspace  VariableName=v_fht_alpha_sim  SampleTime=-1
      settings: MaxDataPoints=glb_time.Ns_afe
  To Workspace5 : ToWorkspace  VariableName=u_fhtsr_alpha_sim  SampleTime=-1
      settings: MaxDataPoints=glb_time.Ns_afe
  To Workspace6 : ToWorkspace  VariableName=u_fhtsr_beta_sim  SampleTime=-1
      settings: MaxDataPoints=glb_time.Ns_afe
  To Workspace7 : ToWorkspace  VariableName=u_fht_beta_sim  SampleTime=-1
      settings: MaxDataPoints=glb_time.Ns_afe
  To Workspace8 : ToWorkspace  VariableName=v_fht_beta_sim  SampleTime=-1
      settings: MaxDataPoints=glb_time.Ns_afe
  To Workspace9 : ToWorkspace  VariableName=ugd_abc_grid_sim  SampleTime=-1
      settings: MaxDataPoints=glb_time.Ns_afe
  abc2alphabeta : MATLAB Function  TreatAsAtomicUnit=on
  grid_voltages : Scope  NumInputPorts=3
      settings: ActiveDisplayYMinimum=-1.3618303835391998  ActiveDisplayYMaximum=1.3331545889377594  DataLoggingVariableName=ScopeData13
  ug_alpha : Outport  VectorParamsAs1DForOutWhenUnconnected=off
  ug_beta : Outport  Port=2  VectorParamsAs1DForOutWhenUnconnected=off
  wires:
  ug_b/1 -> Bus Creator3/2, grid_voltages/2, abc2alphabeta/2(b)  "ugd_b"
  ug_c/1 -> Bus Creator3/3, grid_voltages/3, abc2alphabeta/3(c)  "ugd_c"
  ug_a/1 -> Bus Creator3/1, grid_voltages/1, abc2alphabeta/1(a)  "ugd_a"
  abc2alphabeta/1(alpha) -> To Workspace1/1, FHTalpha/1(u), Bus Creator4/1  "u_grid_alpha"
  abc2alphabeta/2(beta) -> FHTbeta/1(u), To Workspace2/1, Bus Creator1/1  "u_grid_beta"
  FHTalpha/1(ud_hat) -> To Workspace3/1, Bus Creator/1, Sum/1  "u_fht_alpha"
  Sum/1 -> Gain/1
  FHTbeta/1(ud_hat) -> Sum1/2, To Workspace7/1, Bus Creator2/1  "u_fht_beta"
  Sum1/1 -> Gain1/1
  Gain1/1 -> Bus Creator1/3, To Workspace6/1, ug_beta/1  "u_fhtsr_beta"
  Gain/1 -> Bus Creator4/3, To Workspace5/1, ug_alpha/1  "u_fhtsr_alpha"
  FHTbeta/2(uq_hat) -> Sum/2, To Workspace8/1, Bus Creator2/2  "v_fht_beta"
  FHTalpha/2(uq_hat) -> Sum1/1, To Workspace4/1, Bus Creator/2  "v_fht_alpha"
  Bus Creator1/1 -> FHTdqPLL/2
  Bus Creator4/1 -> FHTdqPLL/1
  Bus Creator/1 -> Bus Creator4/2  "FHTalpha"
  Bus Creator2/1 -> Bus Creator1/2  "FHTbeta"
  Bus Creator3/1 -> To Workspace9/1

== system grid_afe_n/afe_abc_mod3/AFE_control/afe_control/grid_voltage_phase_lock_loops/FHT-PLL/pll_stageA/sequences ==
  u_grid_alpha : Inport
  u_grid_beta : Inport  Port=2
  phase_angle : Inport  Port=3
  alphabeta2xieta : MATLAB Function  TreatAsAtomicUnit=on
  u_grid_xi : Outport
  u_grid_eta : Outport  Port=2
  wires:
  alphabeta2xieta/1(xi) -> u_grid_xi/1  "u_grid_xi"
  alphabeta2xieta/2(eta) -> u_grid_eta/1  "u_grid_eta"
  u_grid_alpha/1 -> alphabeta2xieta/1(alpha)  "u_grid_alpha"
  u_grid_beta/1 -> alphabeta2xieta/2(beta)  "u_grid_beta"
  phase_angle/1 -> alphabeta2xieta/3(gamma)  "phase_angle"

== system grid_afe_n/afe_abc_mod3/AFE_control/afe_control/grid_voltage_phase_lock_loops/FHT-PLL/pll_stageB/double_integrator_observer ==
  theta : Inport
  Gain : Gain  Gain=afe_ctrl.di_obs.Ldso  Multiplication=Matrix(K*u)
  Gain1 : Gain  Gain=afe_ctrl.di_obs.Adso  Multiplication=Matrix(K*u)
  Gain2 : Gain  Gain=afe_ctrl.di_obs.Cso  Multiplication=Matrix(K*u)
  Selector : Selector  InputPortWidth=2  IndexOptions=Index vector (dialog)  Indices=2  OutputSizes=1
  Sum : Sum  Inputs=-+|
  Sum1 : Sum  Inputs=|++
  Unit Delay : UnitDelay  SampleTime=-1
  bounder1 : MATLAB Function  TreatAsAtomicUnit=on
  bounder2 : MATLAB Function  TreatAsAtomicUnit=on
  omega_hat : Outport
  wires:
  Gain/1 -> Sum1/1
  Selector/1 -> omega_hat/1
  Gain2/1 -> bounder2/1(u)  "theta_hat"
  Gain1/1 -> Sum1/2
  Sum1/1 -> Unit Delay/1
  Sum/1 -> bounder1/1(u)  "e"
  Unit Delay/1 -> Gain1/1, Selector/1, Gain2/1
  theta/1 -> Sum/2  "theta"
  bounder1/1(y) -> Gain/1
  bounder2/1(y) -> Sum/1  "theta_hat_bounded"

== system grid_afe_n/afe_abc_mod3/AFE_control/afe_control/grid_voltage_phase_lock_loops/FHT-PLL_simulink/pll_stageA/filter_and_transformation ==
  ug_a : Inport
  ug_b : Inport  Port=2
  ug_c : Inport  Port=3
  Bus Creator : BusCreator  Inputs=2
  Bus Creator1 : BusCreator  Inputs=3
  Bus Creator2 : BusCreator  Inputs=2
  Bus Creator4 : BusCreator  Inputs=3
  FHTalpha : Subsystem
  FHTbeta : Subsystem
  FHTdqPLL : Scope  NumInputPorts=2
      settings: ActiveDisplayYMinimum=-1.5258214459194912  ActiveDisplayYMaximum=1.5258228058860459  DataLoggingVariableName=ScopeData12
  Gain : Gain  Gain=-1/2
  Gain1 : Gain  Gain=-1/2
  Sum : Sum  Inputs=|++
  Sum1 : Sum  Inputs=-+|
  abc2alphabeta : MATLAB Function  TreatAsAtomicUnit=on
  grid_voltages : Scope  NumInputPorts=3
      settings: ActiveDisplayYMinimum=-1.3618303835391998  ActiveDisplayYMaximum=1.3331545889377594  DataLoggingVariableName=ScopeData13
  ug_alpha : Outport  VectorParamsAs1DForOutWhenUnconnected=off
  ug_beta : Outport  Port=2  VectorParamsAs1DForOutWhenUnconnected=off
  wires:
  Bus Creator2/1 -> Bus Creator1/2  "FHTbeta"
  Bus Creator/1 -> Bus Creator4/2  "FHTalpha"
  Bus Creator4/1 -> FHTdqPLL/1
  Bus Creator1/1 -> FHTdqPLL/2
  FHTalpha/2(ubeta) -> Bus Creator/2, Sum1/1  "v_fht_alpha"
  FHTbeta/2(ubeta) -> Bus Creator2/2, Sum/2  "v_fht_beta"
  Gain/1 -> ug_alpha/1, Bus Creator4/3  "u_fhtsr_alpha"
  Gain1/1 -> ug_beta/1, Bus Creator1/3  "u_fhtsr_beta"
  Sum1/1 -> Gain1/1
  FHTbeta/1(ualpha) -> Bus Creator2/1, Sum1/2  "u_fht_beta"
  Sum/1 -> Gain/1
  FHTalpha/1(ualpha) -> Sum/1, Bus Creator/1  "u_fht_alpha"
  abc2alphabeta/2(beta) -> FHTbeta/1(u), Bus Creator1/1  "u_grid_beta"
  abc2alphabeta/1(alpha) -> FHTalpha/1(u), Bus Creator4/1  "u_grid_alpha"
  ug_a/1 -> abc2alphabeta/1(a), grid_voltages/1  "ugd_a"
  ug_c/1 -> abc2alphabeta/3(c), grid_voltages/3  "ugd_c"
  ug_b/1 -> abc2alphabeta/2(b), grid_voltages/2  "ugd_b"

== system grid_afe_n/afe_abc_mod3/AFE_control/afe_control/grid_voltage_phase_lock_loops/FHT-PLL_simulink/pll_stageA/sequences ==
  u_grid_alpha : Inport
  u_grid_beta : Inport  Port=2
  phase_angle : Inport  Port=3
  alphabeta2xieta : MATLAB Function  TreatAsAtomicUnit=on
  u_grid_xi : Outport
  u_grid_eta : Outport  Port=2
  wires:
  phase_angle/1 -> alphabeta2xieta/3(gamma)  "phase_angle"
  u_grid_beta/1 -> alphabeta2xieta/2(beta)  "u_grid_beta"
  u_grid_alpha/1 -> alphabeta2xieta/1(alpha)  "u_grid_alpha"
  alphabeta2xieta/2(eta) -> u_grid_eta/1  "u_grid_eta"
  alphabeta2xieta/1(xi) -> u_grid_xi/1  "u_grid_xi"

== system grid_afe_n/afe_abc_mod3/AFE_control/afe_control/grid_voltage_phase_lock_loops/FHT-PLL_simulink/pll_stageB/double_integrator_observer ==
  theta : Inport
  Gain : Gain  Gain=afe_ctrl.di_obs.Ldso  Multiplication=Matrix(K*u)
  Gain1 : Gain  Gain=afe_ctrl.di_obs.Adso  Multiplication=Matrix(K*u)
  Gain2 : Gain  Gain=afe_ctrl.di_obs.Cso  Multiplication=Matrix(K*u)
  Selector : Selector  InputPortWidth=2  IndexOptions=Index vector (dialog)  Indices=2  OutputSizes=1
  Sum : Sum  Inputs=-+|
  Sum1 : Sum  Inputs=|++
  Unit Delay : UnitDelay  SampleTime=-1
  bounder1 : MATLAB Function  TreatAsAtomicUnit=on
  bounder2 : MATLAB Function  TreatAsAtomicUnit=on
  omega_hat : Outport
  wires:
  bounder2/1(y) -> Sum/1  "theta_hat_bounded"
  bounder1/1(y) -> Gain/1
  theta/1 -> Sum/2  "theta"
  Unit Delay/1 -> Gain2/1, Selector/1, Gain1/1
  Sum/1 -> bounder1/1(u)  "e"
  Sum1/1 -> Unit Delay/1
  Gain1/1 -> Sum1/2
  Gain2/1 -> bounder2/1(u)  "theta_hat"
  Selector/1 -> omega_hat/1
  Gain/1 -> Sum1/1

== system grid_afe_n/afe_abc_mod3/AFE_control/afe_control/grid_voltage_phase_lock_loops/dq_pll/pll_stageA/mormalization_and_transformation ==
  ug_a : Inport
  ug_b : Inport  Port=2
  ug_c : Inport  Port=3
  abc2alphabeta : MATLAB Function  TreatAsAtomicUnit=on
  ug_alpha : Outport  VectorParamsAs1DForOutWhenUnconnected=off
  ug_beta : Outport  Port=2  VectorParamsAs1DForOutWhenUnconnected=off
  wires:
  abc2alphabeta/2(beta) -> ug_beta/1  "u_grid_beta"
  abc2alphabeta/1(alpha) -> ug_alpha/1  "u_grid_alpha"
  ug_a/1 -> abc2alphabeta/1(a)
  ug_b/1 -> abc2alphabeta/2(b)
  ug_c/1 -> abc2alphabeta/3(c)

== system grid_afe_n/afe_abc_mod3/AFE_control/afe_control/grid_voltage_phase_lock_loops/dq_pll/pll_stageA/sequences ==
  u_grid_alpha : Inport
  u_grid_beta : Inport  Port=2
  gamma_grid : Inport  Port=3
  alphabeta2xieta : Subsystem
  u_grid_pos_xi : Outport
  u_grid_pos_eta : Outport  Port=2
  wires:
  alphabeta2xieta/1(xi) -> u_grid_pos_xi/1  "u_grid_pos_xi"
  alphabeta2xieta/2(eta) -> u_grid_pos_eta/1  "u_grid_pos_eta"
  u_grid_alpha/1 -> alphabeta2xieta/1(alpha)  "u_grid_alpha"
  u_grid_beta/1 -> alphabeta2xieta/2(beta)  "u_grid_beta"
  gamma_grid/1 -> alphabeta2xieta/3(gamma)  "phase_grid"

== system grid_afe_n/afe_abc_mod3/AFE_control/afe_control/grid_voltage_phase_lock_loops/dq_pll/pll_stageB/double_integrator_observer ==
  phase : Inport
  Gain : Gain  Gain=afe_ctrl.di_obs.Ldso  Multiplication=Matrix(K*u)
  Gain1 : Gain  Gain=afe_ctrl.di_obs.Adso  Multiplication=Matrix(K*u)
  Gain2 : Gain  Gain=afe_ctrl.di_obs.Cso  Multiplication=Matrix(K*u)
  Selector : Selector  InputPortWidth=2  IndexOptions=Index vector (dialog)  Indices=2  OutputSizes=1
  Sum : Sum  Inputs=-+|
  Sum1 : Sum  Inputs=|++
  Unit Delay : UnitDelay  SampleTime=-1
  bounder1 : MATLAB Function  TreatAsAtomicUnit=on
  bounder2 : MATLAB Function  TreatAsAtomicUnit=on
  omega_hat : Outport
  wires:
  Gain/1 -> Sum1/1
  Selector/1 -> omega_hat/1
  Gain2/1 -> bounder2/1(u)  "theta_hat"
  Gain1/1 -> Sum1/2
  Sum1/1 -> Unit Delay/1
  Sum/1 -> bounder1/1(u)  "e"
  Unit Delay/1 -> Gain1/1, Selector/1, Gain2/1
  phase/1 -> Sum/2  "phase"
  bounder1/1(y) -> Gain/1  "e_bounded"
  bounder2/1(y) -> Sum/1  "theta_hat_bounded"

== system grid_afe_n/afe_abc_mod3/AFE_control/afe_control/grid_voltage_phase_lock_loops/dq_pll/pll_stageB/scheduled-p-gain ==
  In1 : Inport
  Switch : Switch  Criteria=u2 > Threshold  Threshold=0.5  SaturateOnIntegerOverflow=off  InputSameDT=off
  kp1 : Gain  Gain=afe_ctrl.pll_p  SaturateOnIntegerOverflow=on  OutDataTypeStr=Inherit: Same as input  ParamDataTypeStr=Inherit: Same as input
  kp3 : Gain  Gain=afe_ctrl.pll_p_frt  SaturateOnIntegerOverflow=on  OutDataTypeStr=Inherit: Same as input  ParamDataTypeStr=Inherit: Same as input
  Out2 : Outport
  wires:
  kp3/1 -> Switch/1
  kp1/1 -> Switch/3
  [frt_active] -> Switch/2
  In1/1 -> kp1/1, kp3/1
  Switch/1 -> Out2/1

== system grid_afe_n/afe_abc_mod4/AFE_control/afe_control/current_ctrl/inner_current_ctrl/zero_current_ctrl/antiwind_up ==
  d_abc : Inport
  Add : Sum
  Bus Creator : BusCreator  Inputs=3
  Constant : Constant  Value=0
  Demux1 : Demux  Outputs=3
  MATLAB Function1 : MATLAB Function  TreatAsAtomicUnit=on
  MATLAB Function2 : MATLAB Function  TreatAsAtomicUnit=on
  Terminator : Terminator
  Unit Delay1 : UnitDelay  SampleTime=-1
  Unit Delay4 : UnitDelay  SampleTime=-1
  Unit Delay5 : UnitDelay  SampleTime=-1
  afe_ictrl_out/afe_ictrl_ff : Scope  NumInputPorts=3
      settings: ActiveDisplayYMinimum=-2.3644997050526393  ActiveDisplayYMaximum=2.3332899605671109  DataLoggingVariableName=ScopeData4
  anti_wind_up : Subsystem
  ualpha_afe : Outport
  ubeta_afe : Outport  Port=2
  wires:
  Constant/1 -> Add/2
  MATLAB Function2/3(gamma) -> Terminator/1  "u_gamma"
  Unit Delay5/1 -> ubeta_afe/1, anti_wind_up/2(beta)  "ubeta_afe"
  MATLAB Function2/2(beta) -> Unit Delay5/1  "u_beta"
  Unit Delay4/1 -> ualpha_afe/1, anti_wind_up/1(alpha)  "ualpha_afe"
  MATLAB Function2/1(alpha) -> Unit Delay4/1  "u_alpha"
  MATLAB Function1/2(dbs) -> Bus Creator/2, MATLAB Function2/2(b)  "dbs"
  Add/1 -> Demux1/1  "d_abc_sum"
  Demux1/1 -> MATLAB Function1/1(da)  "da"
  anti_wind_up/1(scaling) -> MATLAB Function1/4(scaling)
  Unit Delay1/1 -> afe_ictrl_out/afe_ictrl_ff/3  "u_grid_ff_abc_mod1"
  Bus Creator/1 -> afe_ictrl_out/afe_ictrl_ff/1  "ds_abc"
  Demux1/3 -> MATLAB Function1/3(dc)  "dc"
  Demux1/2 -> MATLAB Function1/2(db)  "db"
  [v_grid_ff_abc] -> Unit Delay1/1
  MATLAB Function1/3(dcs) -> Bus Creator/3, MATLAB Function2/3(c)  "dcs"
  d_abc/1 -> afe_ictrl_out/afe_ictrl_ff/2, Add/1
  MATLAB Function1/1(das) -> Bus Creator/1, MATLAB Function2/1(a)  "das"

== system grid_afe_n/afe_abc_mod4/AFE_control/afe_control/current_ctrl/inner_current_ctrl/zero_current_ctrl/iz ==
  Demux : Demux  Outputs=3
  Gain : Gain  Gain=1/3
  Sum : Sum  Inputs=+++
  iz : Outport
  wires:
  Gain/1 -> iz/1
  Demux/2 -> Sum/2  "is_b"
  Demux/3 -> Sum/3  "is_c"
  [isd_abc_pu] -> Demux/1
  Demux/1 -> Sum/1  "is_a"
  Sum/1 -> Gain/1

== system grid_afe_n/afe_abc_mod4/AFE_control/afe_control/current_ctrl/inner_current_ctrl/zero_current_ctrl/zero_sequence_current_ctrl ==
  iz : Inport
  1/Ti : Gain  Gain=afe_ctrl.kp_is_z  SaturateOnIntegerOverflow=on  OutDataTypeStr=Inherit: Same as input  ParamDataTypeStr=Inherit: Same as input
  Constant1 : Constant  Value=0
  Gain : Gain
  Saturation : Saturate  UpperLimit=1  LowerLimit=-1
  Sum1 : Sum  Inputs=+++  SaturateOnIntegerOverflow=on
  Sum2 : Sum  Inputs=-+  SaturateOnIntegerOverflow=on
  Sum3 : Sum  Inputs=-+  SaturateOnIntegerOverflow=on
  Unit Delay4 : UnitDelay  SampleTime=-1
  iz_tracking : Scope  NumInputPorts=3
      settings: ActiveDisplayYMinimum=-1  ActiveDisplayYMaximum=1  DataLoggingVariableName=ScopeData8
  kp : Gain  Gain=afe_ctrl.ki_is_z*glb_time.ts_afe  SaturateOnIntegerOverflow=on  OutDataTypeStr=Inherit: Same as input  ParamDataTypeStr=Inherit: Same as input
  ugamma_afe : Outport
  tag scope: iz_ctrl_out=scoped, iz_pu=scoped, iz_pu_ref=scoped
  wires:
  Gain/1 -> ugamma_afe/1
  Saturation/1 -> Sum3/2, iz_tracking/3, [iz_ctrl_out], Gain/1  "iz_ctrl_out"
  Sum1/1 -> Saturation/1
  Sum2/1 -> 1/Ti/1, kp/1
  iz/1 -> Sum2/1, iz_tracking/2, [iz_pu]  "iz_pu"
  Constant1/1 -> Sum2/2, iz_tracking/1, [iz_pu_ref]  "iz_pu_ref"
  Unit Delay4/1 -> Sum1/3
  Sum3/1 -> Unit Delay4/1
  kp/1 -> Sum1/2
  1/Ti/1 -> Sum3/1, Sum1/1
